simulink model "Energy_Shaping"  (R2022b)
settings: Solver=FixedStepAuto  StartTime=0.0  StopTime=50  FixedStep=0.001  RelTol=1e-3
undefined symbols (not defined in the file): K_LQR, l_v, m_v, M_v, theta_desired
settings Model: Creator=ali14  LastModifiedBy=ali14

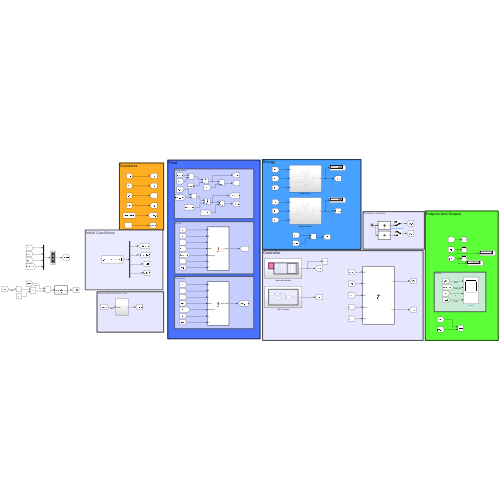
[thumbnail: Simulink's stored preview of the top-level diagram]
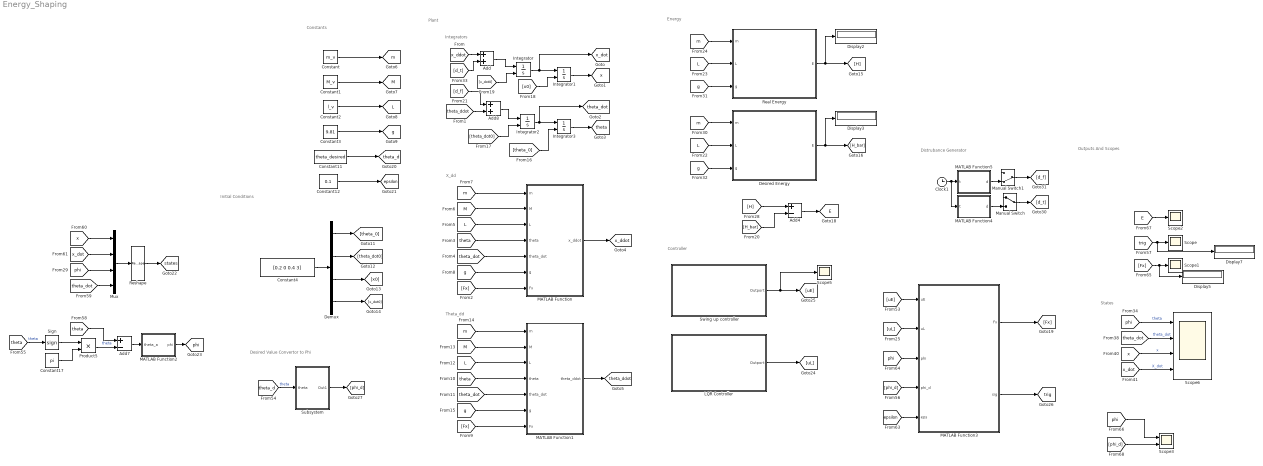
== system Energy_Shaping ==
  note: Controller
  note: States
  note: Outputs And Scopes
  note: Distrubance Generator
  note: Energy
  note: Integrators
  note: Theta_dd
  note: X_dd
  note: Desired Value Convertor to Phi
  note: Initial Conditions
  note: Constants
  note: Plant
  Add : Sum
  Add4 : Sum  Inputs=+-
  Add7 : Sum  Inputs=+-
  Add8 : Sum
  Clock1 : Clock
  Constant : Constant  Value=m_v
  Constant1 : Constant  Value=M_v
  Constant11 : Constant  Value=theta_desired
  Constant12 : Constant  Value=0.1
  Constant17 : Constant  Value=pi
  Constant2 : Constant  Value=l_v
  Constant3 : Constant  Value=9.81
  Constant4 : Constant  Value=[0.2 0 0.4 3]
  Demux : Demux
  Desired Energy : Subsystem
  Display{2..3,5,7} (4 alike) : Display
  Integrator : Integrator  InitialConditionSource=external
  Integrator1 : Integrator  InitialConditionSource=external
  Integrator2 : Integrator  InitialConditionSource=external  UpperSaturationLimit=pi/2  LowerSaturationLimit=-pi/2
  Integrator3 : Integrator  InitialConditionSource=external  UpperSaturationLimit=pi/2  LowerSaturationLimit=-pi/2  WrapState=on
  LQR Controller : Subsystem
  MATLAB Function : MATLAB Function  TreatAsAtomicUnit=on
  MATLAB Function1 : MATLAB Function  TreatAsAtomicUnit=on
  MATLAB Function2 : MATLAB Function  TreatAsAtomicUnit=on
  MATLAB Function3 : MATLAB Function  TreatAsAtomicUnit=on
  MATLAB Function4 : MATLAB Function  TreatAsAtomicUnit=on
  MATLAB Function5 : MATLAB Function  TreatAsAtomicUnit=on
  Manual Switch : ManualSwitch
  Manual Switch1 : ManualSwitch  CurrentSetting=0
  Mux : Mux
  Product5 : Product
  Real Energy : Subsystem
  Reshape : Reshape  OutputDimensionality=Column vector (2-D)
  Scope{,1..2,5} (4 alike) : Scope
  Scope3 : Scope  NumInputPorts=2
  Scope6 : Scope  NumInputPorts=4
  Sign : Signum
  Subsystem : Subsystem
  Swing up controller : Subsystem
  tag scope: E=global, L=global, M=global, epsilon=global, g=global, m=global, phi=global, states=global, theta=global, theta_d=global, theta_ddot=global, theta_dot=global, trig=global, x=global, x_ddot=global, x_dot=global
  wires:
  Integrator/1 -> [x_dot], Integrator1/1
  Integrator1/1 -> [x]
  Integrator3/1 -> [theta]
  Integrator2/1 -> [theta_dot], Integrator3/1
  Constant/1 -> [m]
  Constant1/1 -> [M]
  Constant2/1 -> [L]
  [theta_dot] -> MATLAB Function/5(theta_dot)
  [theta] -> MATLAB Function/4(theta)
  [L] -> MATLAB Function/3(L)
  [M] -> MATLAB Function/2(M)
  [m] -> MATLAB Function/1(m)
  Constant3/1 -> [g]
  [g] -> MATLAB Function/6(g)
  [Fx] -> MATLAB Function/7(Fx)
  [Fx] -> MATLAB Function1/7(Fx)
  [M] -> MATLAB Function1/2(M)
  [theta_dot] -> MATLAB Function1/5(theta_dot)
  [L] -> MATLAB Function1/3(L)
  [theta] -> MATLAB Function1/4(theta)
  [g] -> MATLAB Function1/6(g)
  [m] -> MATLAB Function1/1(m)
  MATLAB Function1/1(theta_ddot) -> [theta_ddot]
  Constant4/1 -> Demux/1
  Demux/1 -> [theta_0]
  Demux/2 -> [theta_dot0]
  Demux/3 -> [x0]
  Demux/4 -> [x_dot0]
  [theta_0] -> Integrator3/2
  [theta_dot0] -> Integrator2/2
  [x0] -> Integrator1/2
  [x_dot0] -> Integrator/2
  MATLAB Function/1(x_ddot) -> [x_ddot]
  [H] -> Add4/1
  [H_bar] -> Add4/2
  Add4/1 -> [E]
  Constant11/1 -> [theta_d]
  [phi] -> MATLAB Function3/3(phi)
  Constant12/1 -> [epsilon]
  Mux/1 -> Reshape/1
  Reshape/1 -> [states]
  [x] -> Mux/1
  [x_dot] -> Mux/2
  [theta_dot] -> Mux/4
  [epsilon] -> MATLAB Function3/5(eps)
  [theta] -> Add7/1  "theta"
  Product5/1 -> Add7/2
  Constant17/1 -> Product5/2
  Sign/1 -> Product5/1
  [theta] -> Sign/1  "theta"
  [uL] -> MATLAB Function3/2(uL)
  [uE] -> MATLAB Function3/1(uE)
  MATLAB Function3/2(sig) -> [trig]
  [phi_d] -> MATLAB Function3/4(phi_d)
  [x_dot] -> Scope6/4  "X_dot"
  [theta_dot] -> Scope6/2  "theta_dot"
  [x] -> Scope6/3  "x"
  [phi] -> Scope6/1  "theta"
  Subsystem/1(Out1) -> [phi_d]
  [theta_d] -> Subsystem/1(theta)  "theta"
  [trig] -> Display7/1, Scope/1
  [Fx] -> Display5/1, Scope1/1
  [E] -> Scope2/1
  MATLAB Function3/1(Fx) -> [Fx]
  [phi] -> Scope3/1
  [phi_d] -> Scope3/2
  Add8/1 -> Integrator2/1
  [theta_ddot] -> Add8/2
  [d_f] -> Add8/1
  Manual Switch/1 -> [d_t]
  MATLAB Function4/1(d) -> Manual Switch/2
  Real Energy/1(E) -> Display2/1, [H]
  [m] -> Real Energy/1(m)
  [L] -> Real Energy/2(L)
  [g] -> Real Energy/3(g)
  [g] -> Desired Energy/3(g)
  [L] -> Desired Energy/2(L)
  Desired Energy/1(E) -> [H_bar], Display3/1
  [m] -> Desired Energy/1(m)
  Manual Switch1/1 -> [d_f]
  Clock1/1 -> MATLAB Function4/1(t), MATLAB Function5/1(t)
  MATLAB Function5/1(d) -> Manual Switch1/2
  Swing up controller/1(Outport) -> Scope5/1, [uE]
  LQR Controller/1(Outport) -> [uL]
  [phi] -> Mux/3
  Add7/1 -> MATLAB Function2/1(theta_a)
  MATLAB Function2/1(phi) -> [phi]
  [x_ddot] -> Add/1
  Add/1 -> Integrator/1
  [d_t] -> Add/2

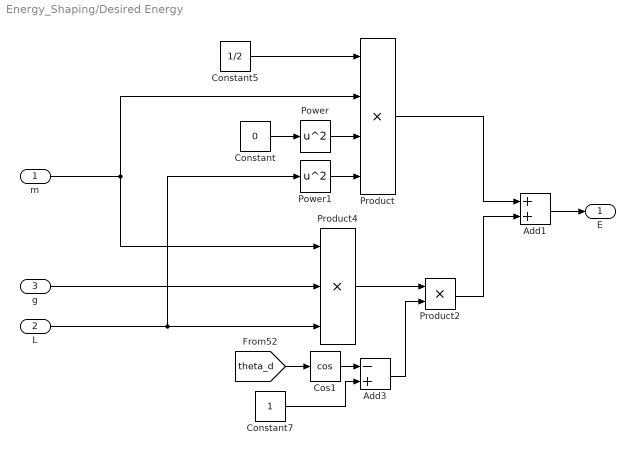
== system Energy_Shaping/Desired Energy ==
  m : Inport
  L : Inport  Port=2
  g : Inport  Port=3
  Add1 : Sum
  Add3 : Sum  Inputs=-+
  Constant : Constant  Value=0
  Constant5 : Constant  Value=1/2
  Constant7 : Constant
  Cos1 : Trigonometry  Operator=cos
  Power : Math  Operator=square
  Power1 : Math  Operator=square
  Product : Product  Inputs=4
  Product2 : Product
  Product4 : Product  Inputs=3
  E : Outport
  wires:
  Product4/1 -> Product2/1
  Power/1 -> Product/3
  Constant7/1 -> Add3/2
  m/1 -> Product4/1, Product/2
  Constant/1 -> Power/1
  Product/1 -> Add1/1
  Cos1/1 -> Add3/1
  Add3/1 -> Product2/2
  Power1/1 -> Product/4
  Product2/1 -> Add1/2
  [theta_d] -> Cos1/1
  Constant5/1 -> Product/1
  Add1/1 -> E/1
  g/1 -> Product4/2
  L/1 -> Power1/1, Product4/3

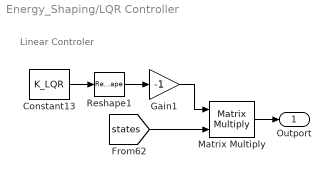
== system Energy_Shaping/LQR Controller ==
  note: Linear Controler
  Constant13 : Constant  Value=K_LQR
  Gain1 : Gain  Gain=-1
  Matrix Multiply : Product  Multiplication=Matrix(*)
  Reshape1 : Reshape  OutputDimensionality=Row vector (2-D)
  Outport : Outport
  wires:
  Reshape1/1 -> Gain1/1
  [states] -> Matrix Multiply/2
  Constant13/1 -> Reshape1/1
  Matrix Multiply/1 -> Outport/1
  Gain1/1 -> Matrix Multiply/1

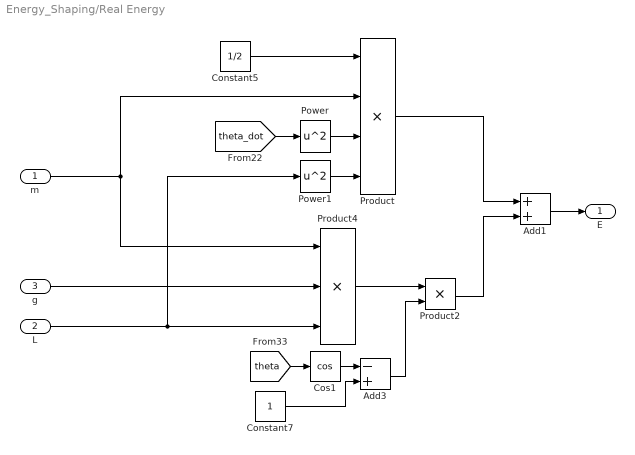
== system Energy_Shaping/Real Energy ==
  m : Inport
  L : Inport  Port=2
  g : Inport  Port=3
  Add1 : Sum
  Add3 : Sum  Inputs=-+
  Constant5 : Constant  Value=1/2
  Constant7 : Constant
  Cos1 : Trigonometry  Operator=cos
  Power : Math  Operator=square
  Power1 : Math  Operator=square
  Product : Product  Inputs=4
  Product2 : Product
  Product4 : Product  Inputs=3
  E : Outport
  wires:
  Product4/1 -> Product2/1
  Power/1 -> Product/3
  Constant7/1 -> Add3/2
  m/1 -> Product4/1, Product/2
  [theta_dot] -> Power/1
  Product/1 -> Add1/1
  Cos1/1 -> Add3/1
  Add3/1 -> Product2/2
  Power1/1 -> Product/4
  Product2/1 -> Add1/2
  [theta] -> Cos1/1
  Constant5/1 -> Product/1
  Add1/1 -> E/1
  g/1 -> Product4/2
  L/1 -> Power1/1, Product4/3

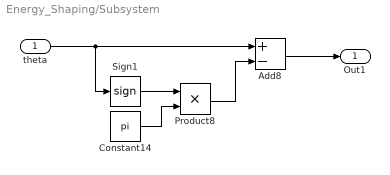
== system Energy_Shaping/Subsystem ==
  theta : Inport
  Add8 : Sum  Inputs=+-
  Constant14 : Constant  Value=pi
  Product8 : Product
  Sign1 : Signum
  Out1 : Outport
  wires:
  Product8/1 -> Add8/2
  theta/1 -> Add8/1, Sign1/1
  Constant14/1 -> Product8/2
  Sign1/1 -> Product8/1
  Add8/1 -> Out1/1

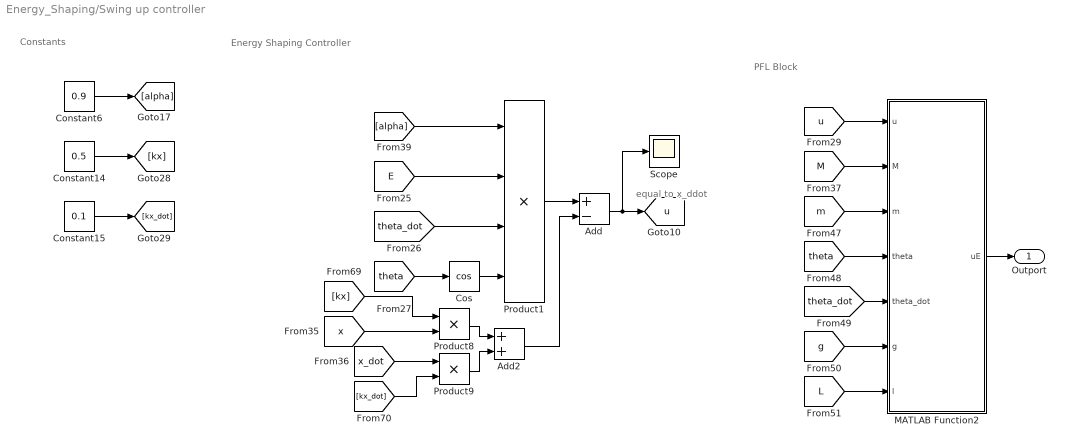
== system Energy_Shaping/Swing up controller ==
  note: PFL Block
  note: equal to x_ddot
  note: Constants
  note: Energy Shaping Controller
  Add : Sum  Inputs=+-
  Add2 : Sum
  Constant14 : Constant  Value=0.5
  Constant15 : Constant  Value=0.1
  Constant6 : Constant  Value=0.9
  Cos : Trigonometry  Operator=cos
  MATLAB Function2 : MATLAB Function  TreatAsAtomicUnit=on
  Product1 : Product  Inputs=4
  Product8 : Product
  Product9 : Product
  Scope : Scope
  Outport : Outport
  tag scope: u=global
  wires:
  [theta_dot] -> MATLAB Function2/5(theta_dot)
  Add/1 -> Scope/1, [u]
  [M] -> MATLAB Function2/2(M)
  [theta] -> Cos/1
  Product8/1 -> Add2/1
  Product9/1 -> Add2/2
  [theta] -> MATLAB Function2/4(theta)
  [kx] -> Product8/1
  [kx_dot] -> Product9/2
  Cos/1 -> Product1/4
  Constant6/1 -> [alpha]
  Product1/1 -> Add/1
  [u] -> MATLAB Function2/1(u)
  [L] -> MATLAB Function2/7(l)
  [x_dot] -> Product9/1
  [theta_dot] -> Product1/3
  [E] -> Product1/2
  [alpha] -> Product1/1
  Add2/1 -> Add/2
  [x] -> Product8/2
  [g] -> MATLAB Function2/6(g)
  [m] -> MATLAB Function2/3(m)
  MATLAB Function2/1(uE) -> Outport/1
  Constant14/1 -> [kx]
  Constant15/1 -> [kx_dot]

== matlab function Energy_Shaping/MATLAB Function1 ==
  data: m input; theta_ddot output; M input; L input; theta input; theta_dot input; g input; Fx input
function theta_ddot = fcn(m,M,L,theta,theta_dot,g,Fx)

num = m*L*sin(theta)*cos(theta)*theta_dot^2 + ...
       (M+m)*g*sin(theta) + cos(theta)*Fx;

den = (M + m*sin(theta)^2)*L;

theta_ddot = -num/den;

== matlab function Energy_Shaping/MATLAB Function ==
  data: m input; x_ddot output; M input; L input; theta input; theta_dot input; g input; Fx input
function x_ddot = fcn(m,M,L,theta,theta_dot,g,Fx)

num = m*L*sin(theta)*theta_dot^2 + m*g*sin(theta)*cos(theta) + Fx;
den = M + m*sin(theta)^2;

x_ddot = num/den;

== matlab function Energy_Shaping/Swing up controller/MATLAB Function2 ==
  data: u input; uE output; M input; m input; theta input; theta_dot input; g input; l input
function uE = fcn(u , M ,m ,theta,theta_dot,g,l)

uE = u*(M+m*sin(theta)^2) - ...
(m*l*sin(theta)*theta_dot^2 + m*g*sin(theta)*cos(theta));

== matlab function Energy_Shaping/MATLAB Function3 ==
  settings: updateMethod=DISCRETE
  data: uE input; uL input; phi input; phi_d input; Fx output; eps input; sig output
function [Fx,sig] = fcn(uE, uL, phi, phi_d , eps)

if and(phi > phi_d - eps , phi < phi_d + eps)
    sig = 1;
    Fx = uL;
else
    sig = 0;
    Fx = uE;
end

== matlab function Energy_Shaping/MATLAB Function4 ==
  data: t input; d output
function d = fcn(t)
if and(t > 20 , t <30)
    d = 2 + 4*sin(10*t);
else
    d = 0;
end

== matlab function Energy_Shaping/MATLAB Function5 ==
  data: t input; d output
function d = fcn(t)
if and(t > 20 , t <22)
    d = 2;
else
    d = 0;
end

== matlab function Energy_Shaping/MATLAB Function2 ==
  data: theta_a input; phi output
function phi = fcn(theta_a)
if theta_a == 0
    phi = pi;
else
    phi = theta_a;
end
